simulink model "LunarMicrogrid_Full_Arch"  (R2026b)
settings: Solver=ode23t  StopTime=simulation.timeSim  MaxStep=1/(5*solarPlant.converterSwitchingFrequency)  AbsTol=1e-3
PreLoadFcn:
  | run('LunarMicrogridA_Data');
values from neighbouring files (symbols this model uses):
  Csc = Csc_cell/Ns_sc*Np_sc    (= 200)    [LunarDAB_Params.m]
  eta_sc = 0.95    [LunarDAB_Params.m]
  fsw = 100e3    (= 100000)    [LunarDAB_Params.m]
  k_restore = 1    [LunarDAB_Params.m]
  kiCurrent = 2    [LunarDAB_Params.m]
  kiVoltage = 8    [LunarDAB_Params.m]
  kpCurrent = 0.005    [LunarDAB_Params.m]
  kpVoltage = 0.4    [LunarDAB_Params.m]
  lTotal = lSeries + Llk    [LunarDAB_Params.m]
  P170_dt = 1e-4    (= 0.0001)    [P170_PV_Initialize.m]
  P170_Imp = im(ix)    [P170_PV_Initialize.m]
  P170_Vmp = vm(ix)    [P170_PV_Initialize.m]
  Rd_bat = dV_droop/Ibat_max    (= 0.232258064516)    [LunarDAB_Params.m]
  SC_enable = 1    [LunarDAB_Params.m]
  thetaIC = 0    [LunarDAB_Params.m]
  thetaMaxDab = pi/4    (= 0.785398163397)    [LunarDAB_Params.m]
  Tsw = 1/fsw    (= 1e-05)    [LunarDAB_Params.m]
  Vsc0 = sqrt((Vsc_max^2 + Vsc_min^2)/2)    [LunarDAB_Params.m]
  Vsc_max = 119    [LunarDAB_Params.m]
  Vsc_min = 66    [LunarDAB_Params.m]
undefined symbols (not defined in the file or in its folder): a_lpf_sys, battery, bms, connectedLoad, dcVoltage, DiscIntNeverNeededParam, eta_dab, Ibat_sign, mmc, Ndab, P170_T, pvDroop, sc, sensor, socLimit, solarPlant
libraries: sl_discontinuities x13, fl_lib x13, nesl_utility x13, simulink x7, batteryecm_lib x1, simulink_extras x1, ee_lib x1
(part 6 of 8)

== system LunarMicrogrid_Full_Arch/Battery + DAB + Supercap/BESS Controller/DABCtrl2/Ideal P Gain Fdbk/Internal Parameters ==
  In1 : Inport  SampleTime=SampleTime
  P Gain : Inport  Port=2  SampleTime=SampleTime
  Proportional Gain : Gain  Gain=P  ParamMin=PParamMin  ParamMax=PParamMax  OutMin=POutMin  OutMax=POutMax  RndMeth=Simplest  OutDataTypeStr=Inherit: Same as input
  Signal Specification1 : SignalSpecification  DisableCoverage=on  OutDataTypeStr=boolean  SampleTime=SampleTime
  Terminator1 : Terminator
  Out1 : Outport  SampleTime=SampleTime
  wires:
  Proportional Gain/1 -> Out1/1
  In1/1 -> Proportional Gain/1
  Signal Specification1/1 -> Terminator1/1
  P Gain/1 -> Signal Specification1/1

== system LunarMicrogrid_Full_Arch/Battery + DAB + Supercap/BESS Controller/DABCtrl2/Ideal P Gain Fdbk/Passthrough ==
  In1 : Inport  SampleTime=SampleTime
  P Gain : Inport  Port=2  SampleTime=SampleTime
  Terminator1 : Terminator
  Out1 : Outport  SampleTime=SampleTime
  wires:
  In1/1 -> Out1/1
  P Gain/1 -> Terminator1/1

== system LunarMicrogrid_Full_Arch/Battery + DAB + Supercap/BESS Controller/DABCtrl2/Integrator/Continuous ==
  U : Inport  SampleTime=SampleTime
  Reset : Inport  Port=2  SampleTime=SampleTime
  I0in : Inport  Port=3  SampleTime=SampleTime
  Ground : Ground  DisableCoverage=on
  Integrator : Integrator
  Signal Specification1 : SignalSpecification  DisableCoverage=on  OutDataTypeStr=boolean  SampleTime=SampleTime
  Terminator : Terminator
  Terminator1 : Terminator
  state : Outport  SampleTime=SampleTime
  out : Outport  Port=2  SampleTime=SampleTime
  wires:
  U/1 -> Integrator/1
  I0in/1 -> Terminator/1
  Integrator/1 -> out/1
  Ground/1 -> Signal Specification1/1
  Signal Specification1/1 -> state/1
  Reset/1 -> Terminator1/1

== system LunarMicrogrid_Full_Arch/Battery + DAB + Supercap/BESS Controller/DABCtrl2/Integrator/Disabled ==
  U : Inport  SampleTime=SampleTime
  Reset : Inport  Port=2  SampleTime=SampleTime
  I0in : Inport  Port=3  SampleTime=SampleTime
  Ground : Ground  DisableCoverage=on
  Signal Specification1 : SignalSpecification  DisableCoverage=on  OutDataTypeStr=boolean  SampleTime=SampleTime
  Signal Specification2 : SignalSpecification  DisableCoverage=on  OutDataTypeStr=boolean  SampleTime=SampleTime
  Signal Specification4 : SignalSpecification  DisableCoverage=on  OutDataTypeStr=boolean  SampleTime=SampleTime
  Terminator1 : Terminator
  Terminator2 : Terminator
  Terminator3 : Terminator
  out : Outport  SampleTime=SampleTime
  wires:
  Reset/1 -> Terminator2/1
  Signal Specification4/1 -> Terminator1/1
  I0in/1 -> Signal Specification4/1
  U/1 -> Signal Specification1/1
  Signal Specification1/1 -> Terminator3/1
  Ground/1 -> Signal Specification2/1
  Signal Specification2/1 -> out/1

== system LunarMicrogrid_Full_Arch/Battery + DAB + Supercap/BESS Controller/DABCtrl2/Integrator/Discrete ==
  U : Inport  SampleTime=SampleTime
  Reset : Inport  Port=2  SampleTime=SampleTime
  I0in : Inport  Port=3  SampleTime=SampleTime
  Ground_Integrator : Ground  DisableCoverage=on
  Integrator : DiscreteIntegrator  InitialCondition=thetaIC  SampleTime=SampleTime  OutMin=IntegratorOutMin  OutMax=IntegratorOutMax  RndMeth=Simplest  ICPrevOutput=DiscIntNeverNeededParam  ICPrevScaledInput=DiscIntNeverNeededParam
  Signal Specification1 : SignalSpecification  DisableCoverage=on  OutDataTypeStr=boolean  SampleTime=SampleTime
  Terminator : Terminator
  Terminator1 : Terminator
  Terminator2 : Terminator
  out : Outport  SampleTime=SampleTime
  state : Outport  Port=2  SampleTime=SampleTime
  wires:
  I0in/1 -> Terminator1/1
  Integrator/1 -> out/1
  U/1 -> Integrator/1
  Ground_Integrator/1 -> state/1, Signal Specification1/1
  Signal Specification1/1 -> Terminator/1
  Reset/1 -> Terminator2/1

== system LunarMicrogrid_Full_Arch/Battery + DAB + Supercap/BESS Controller/DABCtrl2/Integrator ICs/Disabled ==
  I0 : Inport  SampleTime=SampleTime
  Ground : Ground  DisableCoverage=on
  Signal Specification : SignalSpecification  DisableCoverage=on  OutDataTypeStr=boolean  SampleTime=SampleTime
  Signal Specification1 : SignalSpecification  DisableCoverage=on  OutDataTypeStr=boolean  SampleTime=SampleTime
  Terminator : Terminator
  Out1 : Outport  SampleTime=SampleTime
  wires:
  Signal Specification/1 -> Terminator/1
  I0/1 -> Signal Specification/1
  Signal Specification1/1 -> Out1/1
  Ground/1 -> Signal Specification1/1

== system LunarMicrogrid_Full_Arch/Battery + DAB + Supercap/BESS Controller/DABCtrl2/Integrator ICs/External IC ==
  I0 : Inport  SampleTime=SampleTime
  Out1 : Outport  SampleTime=SampleTime
  wires:
  I0/1 -> Out1/1

== system LunarMicrogrid_Full_Arch/Battery + DAB + Supercap/BESS Controller/DABCtrl2/Integrator ICs/Internal IC ==
  I0 : Inport  SampleTime=SampleTime
  Ground : Ground  DisableCoverage=on
  Signal Specification : SignalSpecification  DisableCoverage=on  OutDataTypeStr=boolean  SampleTime=SampleTime
  Signal Specification1 : SignalSpecification  DisableCoverage=on  OutDataTypeStr=boolean  SampleTime=SampleTime
  Terminator : Terminator
  Out1 : Outport  SampleTime=SampleTime
  wires:
  I0/1 -> Signal Specification/1
  Signal Specification/1 -> Terminator/1
  Ground/1 -> Signal Specification1/1
  Signal Specification1/1 -> Out1/1

== system LunarMicrogrid_Full_Arch/Battery + DAB + Supercap/BESS Controller/DABCtrl2/N Copy/Disabled ==
  N Gain : Inport  SampleTime=SampleTime
  Terminator : Terminator
  wires:
  N Gain/1 -> Terminator/1

== system LunarMicrogrid_Full_Arch/Battery + DAB + Supercap/BESS Controller/DABCtrl2/N Copy/Disabled wSignal Specification ==
  N Gain : Inport  SampleTime=SampleTime
  Signal Specification1 : SignalSpecification  DisableCoverage=on  OutDataTypeStr=boolean  SampleTime=SampleTime
  Terminator : Terminator
  wires:
  N Gain/1 -> Signal Specification1/1
  Signal Specification1/1 -> Terminator/1

== system LunarMicrogrid_Full_Arch/Battery + DAB + Supercap/BESS Controller/DABCtrl2/N Copy/External Parameters ==
  N Gain : Inport  SampleTime=SampleTime
  Out1 : Outport  SampleTime=SampleTime
  wires:
  N Gain/1 -> Out1/1

== system LunarMicrogrid_Full_Arch/Battery + DAB + Supercap/BESS Controller/DABCtrl2/N Copy/Internal Parameters ==
  N Gain : Inport  SampleTime=SampleTime
  N Copy : Constant  DisableCoverage=on  Value=N  OutMin=NCopyOutMin  OutMax=NCopyOutMax  OutDataTypeStr=Inherit: Inherit via back propagation  PreserveConstantTs=on
  Signal Specification : SignalSpecification  DisableCoverage=on  OutDataTypeStr=boolean  SampleTime=SampleTime
  Terminator : Terminator
  Out1 : Outport  SampleTime=SampleTime
  wires:
  N Copy/1 -> Out1/1
  N Gain/1 -> Signal Specification/1
  Signal Specification/1 -> Terminator/1

== system LunarMicrogrid_Full_Arch/Battery + DAB + Supercap/BESS Controller/DABCtrl2/N Gain/Disabled ==
  U : Inport  SampleTime=SampleTime
  N Gain : Inport  Port=2  SampleTime=SampleTime
  Signal Specification1 : SignalSpecification  DisableCoverage=on  OutDataTypeStr=boolean  SampleTime=SampleTime
  Signal Specification2 : SignalSpecification  DisableCoverage=on  OutDataTypeStr=boolean  SampleTime=SampleTime
  Terminator1 : Terminator
  Terminator2 : Terminator
  wires:
  Signal Specification2/1 -> Terminator2/1
  U/1 -> Signal Specification2/1
  N Gain/1 -> Signal Specification1/1
  Signal Specification1/1 -> Terminator1/1

== system LunarMicrogrid_Full_Arch/Battery + DAB + Supercap/BESS Controller/DABCtrl2/N Gain/External Parameters ==
  U : Inport  SampleTime=SampleTime
  N Gain : Inport  Port=2  SampleTime=SampleTime
  NProd Out : Product  OutMin=NOutMin  OutMax=NOutMax  RndMeth=Simplest  SampleTime=SampleTime
  Out1 : Outport  SampleTime=SampleTime
  wires:
  U/1 -> NProd Out/1
  N Gain/1 -> NProd Out/2
  NProd Out/1 -> Out1/1

== system LunarMicrogrid_Full_Arch/Battery + DAB + Supercap/BESS Controller/DABCtrl2/N Gain/Internal Parameters ==
  U : Inport  SampleTime=SampleTime
  N Gain : Inport  Port=2  SampleTime=SampleTime
  Filter Coefficient : Gain  Gain=N  ParamMin=NParamMin  ParamMax=NParamMax  OutMin=NOutMin  OutMax=NOutMax  RndMeth=Simplest
  Signal Specification1 : SignalSpecification  DisableCoverage=on  OutDataTypeStr=boolean  SampleTime=SampleTime
  Terminator1 : Terminator
  Out1 : Outport  SampleTime=SampleTime
  wires:
  U/1 -> Filter Coefficient/1
  Filter Coefficient/1 -> Out1/1
  N Gain/1 -> Signal Specification1/1
  Signal Specification1/1 -> Terminator1/1

== system LunarMicrogrid_Full_Arch/Battery + DAB + Supercap/BESS Controller/DABCtrl2/N Gain/Passthrough ==
  U : Inport  SampleTime=SampleTime
  N Gain : Inport  Port=2  SampleTime=SampleTime
  Terminator1 : Terminator
  Out1 : Outport  SampleTime=SampleTime
  wires:
  U/1 -> Out1/1
  N Gain/1 -> Terminator1/1

== system LunarMicrogrid_Full_Arch/Battery + DAB + Supercap/BESS Controller/DABCtrl2/P Copy/Disabled ==
  P Gain : Inport  SampleTime=SampleTime
  Terminator3 : Terminator
  wires:
  P Gain/1 -> Terminator3/1

== system LunarMicrogrid_Full_Arch/Battery + DAB + Supercap/BESS Controller/DABCtrl2/P Copy/External Parameters Ideal ==
  P Gain : Inport  SampleTime=SampleTime
  Out1 : Outport  SampleTime=SampleTime
  wires:
  P Gain/1 -> Out1/1

== system LunarMicrogrid_Full_Arch/Battery + DAB + Supercap/BESS Controller/DABCtrl2/P Copy/Internal Parameters Ideal ==
  P Gain : Inport  SampleTime=SampleTime
  P Copy : Constant  DisableCoverage=on  Value=P  OutMin=PCopyOutMin  OutMax=PCopyOutMax  OutDataTypeStr=Inherit: Inherit via back propagation  PreserveConstantTs=on
  Terminator3 : Terminator
  Out1 : Outport  SampleTime=SampleTime
  wires:
  P Copy/1 -> Out1/1
  P Gain/1 -> Terminator3/1

== system LunarMicrogrid_Full_Arch/Battery + DAB + Supercap/BESS Controller/DABCtrl2/Parallel P Gain/Disabled ==
  P Gain : Inport  SampleTime=SampleTime
  Signal Specification : SignalSpecification  DisableCoverage=on  OutDataTypeStr=boolean  SampleTime=SampleTime
  Terminator : Terminator
  wires:
  P Gain/1 -> Signal Specification/1
  Signal Specification/1 -> Terminator/1

== system LunarMicrogrid_Full_Arch/Battery + DAB + Supercap/BESS Controller/DABCtrl2/Parallel P Gain/External Parameters ==
  err : Inport  SampleTime=SampleTime
  P Gain : Inport  Port=2  SampleTime=SampleTime
  PProd Out : Product  OutMin=POutMin  OutMax=POutMax  RndMeth=Simplest  SampleTime=SampleTime  OutDataTypeStr=Inherit: Same as first input
  Out1 : Outport  SampleTime=SampleTime
  wires:
  PProd Out/1 -> Out1/1
  P Gain/1 -> PProd Out/2
  err/1 -> PProd Out/1

== system LunarMicrogrid_Full_Arch/Battery + DAB + Supercap/BESS Controller/DABCtrl2/Parallel P Gain/Internal Parameters ==
  err : Inport  SampleTime=SampleTime
  P Gain : Inport  Port=2  SampleTime=SampleTime
  Proportional Gain : Gain  Gain=P  ParamMin=PParamMin  ParamMax=PParamMax  OutMin=POutMin  OutMax=POutMax  RndMeth=Simplest  OutDataTypeStr=Inherit: Same as input
  Signal Specification : SignalSpecification  DisableCoverage=on  OutDataTypeStr=boolean  SampleTime=SampleTime
  Terminator : Terminator
  Out1 : Outport  SampleTime=SampleTime
  wires:
  Proportional Gain/1 -> Out1/1
  err/1 -> Proportional Gain/1
  Signal Specification/1 -> Terminator/1
  P Gain/1 -> Signal Specification/1

== system LunarMicrogrid_Full_Arch/Battery + DAB + Supercap/BESS Controller/DABCtrl2/Parallel P Gain/Passthrough ==
  err : Inport  SampleTime=SampleTime
  P Gain : Inport  Port=2  SampleTime=SampleTime
  Terminator : Terminator
  Out1 : Outport  SampleTime=SampleTime
  wires:
  err/1 -> Out1/1
  P Gain/1 -> Terminator/1

== system LunarMicrogrid_Full_Arch/Battery + DAB + Supercap/BESS Controller/DABCtrl2/Reset Signal/Disabled ==
  Reset : Inport  SampleTime=SampleTime
  Ground : Ground  DisableCoverage=on
  Signal Specification : SignalSpecification  DisableCoverage=on  OutDataTypeStr=boolean  SampleTime=SampleTime
  Signal Specification1 : SignalSpecification  DisableCoverage=on  OutDataTypeStr=boolean  SampleTime=SampleTime
  Terminator : Terminator
  Out1 : Outport  SampleTime=SampleTime
  wires:
  Reset/1 -> Signal Specification/1
  Signal Specification/1 -> Terminator/1
  Ground/1 -> Signal Specification1/1
  Signal Specification1/1 -> Out1/1

== system LunarMicrogrid_Full_Arch/Battery + DAB + Supercap/BESS Controller/DABCtrl2/Reset Signal/External Reset ==
  Reset : Inport  SampleTime=SampleTime
  Out1 : Outport  SampleTime=SampleTime
  wires:
  Reset/1 -> Out1/1

== system LunarMicrogrid_Full_Arch/Battery + DAB + Supercap/BESS Controller/DABCtrl2/Saturation/Enabled ==
  In1 : Inport  SampleTime=SampleTime
  Upper Limit : Inport  Port=2  SampleTime=SampleTime
  Lower Limit : Inport  Port=3  SampleTime=SampleTime
  Saturation : Saturate  UpperLimit=UpperSaturationLimit  LowerLimit=LowerSaturationLimit  LinearizeAsGain=off  SampleTime=SampleTime  OutMin=SaturationOutMin  OutMax=SaturationOutMax  OutDataTypeStr=Inherit: Inherit via back propagation  RndMeth=Simplest
  Signal Specification : SignalSpecification  DisableCoverage=on  OutDataTypeStr=boolean  SampleTime=SampleTime
  Signal Specification1 : SignalSpecification  DisableCoverage=on  OutDataTypeStr=boolean  SampleTime=SampleTime
  Terminator : Terminator
  Terminator1 : Terminator
  Out1 : Outport  SampleTime=SampleTime
  wires:
  Signal Specification1/1 -> Terminator1/1
  Upper Limit/1 -> Signal Specification/1
  Lower Limit/1 -> Signal Specification1/1
  Signal Specification/1 -> Terminator/1
  In1/1 -> Saturation/1
  Saturation/1 -> Out1/1

== system LunarMicrogrid_Full_Arch/Battery + DAB + Supercap/BESS Controller/DABCtrl2/Saturation/External ==
  In1 : Inport  SampleTime=SampleTime
  Upper Limit : Inport  Port=2  SampleTime=SampleTime
  Lower Limit : Inport  Port=3  SampleTime=SampleTime
  Saturation Dynamic : sl_discontinuities/Saturation Dynamic  OutMin=SaturationOutMin  OutMax=SaturationOutMax  OutDataTypeStr=Inherit: Same as second input  OutDataType=fixdt(1, 16)  OutScaling=2^-10  RndMeth=Simplest  DoSatur=off
  Out1 : Outport  SampleTime=SampleTime
  wires:
  Lower Limit/1 -> Saturation Dynamic/3
  Upper Limit/1 -> Saturation Dynamic/1
  Saturation Dynamic/1 -> Out1/1
  In1/1 -> Saturation Dynamic/2

== system LunarMicrogrid_Full_Arch/Battery + DAB + Supercap/BESS Controller/DABCtrl2/Saturation/Passthrough ==
  In1 : Inport  SampleTime=SampleTime
  Upper Limit : Inport  Port=2  SampleTime=SampleTime
  Lower Limit : Inport  Port=3  SampleTime=SampleTime
  Signal Specification : SignalSpecification  DisableCoverage=on  OutDataTypeStr=boolean  SampleTime=SampleTime
  Signal Specification1 : SignalSpecification  DisableCoverage=on  OutDataTypeStr=boolean  SampleTime=SampleTime
  Terminator : Terminator
  Terminator1 : Terminator
  Out1 : Outport  SampleTime=SampleTime
  wires:
  Signal Specification1/1 -> Terminator1/1
  Lower Limit/1 -> Signal Specification1/1
  Upper Limit/1 -> Signal Specification/1
  Signal Specification/1 -> Terminator/1
  In1/1 -> Out1/1

== system LunarMicrogrid_Full_Arch/Battery + DAB + Supercap/BESS Controller/DABCtrl2/Saturation Fdbk/Disabled ==
  In1 : Inport  SampleTime=SampleTime
  Signal Specification1 : SignalSpecification  DisableCoverage=on  OutDataTypeStr=boolean  SampleTime=SampleTime
  Terminator1 : Terminator
  wires:
  In1/1 -> Signal Specification1/1
  Signal Specification1/1 -> Terminator1/1

== system LunarMicrogrid_Full_Arch/Battery + DAB + Supercap/BESS Controller/DABCtrl2/Saturation Fdbk/Enabled ==
  In1 : Inport  SampleTime=SampleTime
  Saturation : Saturate  UpperLimit=UpperSaturationLimit  LowerLimit=LowerSaturationLimit  LinearizeAsGain=off  SampleTime=SampleTime  OutMin=SaturationOutMin  OutMax=SaturationOutMax  OutDataTypeStr=Inherit: Inherit via back propagation  RndMeth=Simplest
  Out1 : Outport  SampleTime=SampleTime
  wires:
  Saturation/1 -> Out1/1
  In1/1 -> Saturation/1

== system LunarMicrogrid_Full_Arch/Battery + DAB + Supercap/BESS Controller/DABCtrl2/Saturation Fdbk/External ==
  In1 : Inport  SampleTime=SampleTime
  Upper Limit : Inport  Port=2  SampleTime=SampleTime
  Lower Limit : Inport  Port=3  SampleTime=SampleTime
  Saturation Dynamic : sl_discontinuities/Saturation Dynamic  OutMin=SaturationOutMin  OutMax=SaturationOutMax  OutDataTypeStr=Inherit: Same as second input  OutDataType=fixdt(1, 16)  OutScaling=2^-10  RndMeth=Simplest  DoSatur=off
  Out1 : Outport  SampleTime=SampleTime
  wires:
  Lower Limit/1 -> Saturation Dynamic/3
  Upper Limit/1 -> Saturation Dynamic/1
  Saturation Dynamic/1 -> Out1/1
  In1/1 -> Saturation Dynamic/2

== system LunarMicrogrid_Full_Arch/Battery + DAB + Supercap/BESS Controller/DABCtrl2/Saturation Fdbk/Passthrough ==
  In1 : Inport  SampleTime=SampleTime
  Out1 : Outport  SampleTime=SampleTime
  wires:
  In1/1 -> Out1/1

== system LunarMicrogrid_Full_Arch/Battery + DAB + Supercap/BESS Controller/DABCtrl2/Sum/Passthrough_I ==
  P : Inport  SampleTime=SampleTime
  I : Inport  Port=2  SampleTime=SampleTime
  Signal Specification : SignalSpecification  OutDataTypeStr=boolean  SampleTime=SampleTime
  Terminator : Terminator
  Out1 : Outport  SampleTime=SampleTime
  wires:
  Signal Specification/1 -> Terminator/1
  P/1 -> Signal Specification/1
  I/1 -> Out1/1

== system LunarMicrogrid_Full_Arch/Battery + DAB + Supercap/BESS Controller/DABCtrl2/Sum/Passthrough_P ==
  P : Inport  SampleTime=SampleTime
  Out1 : Outport  SampleTime=SampleTime
  wires:
  P/1 -> Out1/1

== system LunarMicrogrid_Full_Arch/Battery + DAB + Supercap/BESS Controller/DABCtrl2/Sum/Sum_PD ==
  P : Inport  SampleTime=SampleTime
  D : Inport  Port=2  SampleTime=SampleTime
  Sum : Sum  Inputs=|++  OutMin=SumOutMin  OutMax=SumOutMax  RndMeth=Simplest  OutDataTypeStr=Inherit: Same as first input
  Out1 : Outport  SampleTime=SampleTime
  wires:
  P/1 -> Sum/1
  D/1 -> Sum/2
  Sum/1 -> Out1/1

== system LunarMicrogrid_Full_Arch/Battery + DAB + Supercap/BESS Controller/DABCtrl2/Sum/Sum_PI ==
  P : Inport  SampleTime=SampleTime
  I : Inport  Port=2  SampleTime=SampleTime
  Sum : Sum  Inputs=|++  OutMin=SumOutMin  OutMax=SumOutMax  RndMeth=Simplest  OutDataTypeStr=Inherit: Same as first input
  Out1 : Outport  SampleTime=SampleTime
  wires:
  I/1 -> Sum/2
  P/1 -> Sum/1
  Sum/1 -> Out1/1

== system LunarMicrogrid_Full_Arch/Battery + DAB + Supercap/BESS Controller/DABCtrl2/Sum/Sum_PID ==
  P : Inport  SampleTime=SampleTime
  I : Inport  Port=2  SampleTime=SampleTime
  D : Inport  Port=3  SampleTime=SampleTime
  Sum : Sum  Inputs=+++  OutMin=SumOutMin  OutMax=SumOutMax  RndMeth=Simplest  OutDataTypeStr=Inherit: Same as first input
  Out1 : Outport  SampleTime=SampleTime
  wires:
  I/1 -> Sum/2
  P/1 -> Sum/1
  D/1 -> Sum/3
  Sum/1 -> Out1/1

== system LunarMicrogrid_Full_Arch/Battery + DAB + Supercap/BESS Controller/DABCtrl2/Sum Fdbk/Disabled ==
  fromP : Inport  SampleTime=SampleTime
  fromState : Inport  Port=2  SampleTime=SampleTime
  fromD : Inport  Port=3  SampleTime=SampleTime
  Signal Specification1 : SignalSpecification  DisableCoverage=on  OutDataTypeStr=boolean  SampleTime=SampleTime
  Terminator1 : Terminator
  Terminator2 : Terminator
  Terminator3 : Terminator
  wires:
  fromD/1 -> Terminator3/1
  fromState/1 -> Signal Specification1/1
  fromP/1 -> Terminator1/1
  Signal Specification1/1 -> Terminator2/1

== system LunarMicrogrid_Full_Arch/Battery + DAB + Supercap/BESS Controller/DABCtrl2/Sum Fdbk/Enabled ==
  fromP : Inport  SampleTime=SampleTime
  fromState : Inport  Port=2  SampleTime=SampleTime
  fromD : Inport  Port=3  SampleTime=SampleTime
  Sum Fdbk : Sum  DisableCoverage=on  Inputs=+++  OutMin=SumOutMin  OutMax=SumOutMax  RndMeth=Simplest  OutDataTypeStr=Inherit: Same as first input
  Out1 : Outport  SampleTime=SampleTime
  wires:
  fromP/1 -> Sum Fdbk/1
  fromState/1 -> Sum Fdbk/2
  fromD/1 -> Sum Fdbk/3
  Sum Fdbk/1 -> Out1/1

== system LunarMicrogrid_Full_Arch/Battery + DAB + Supercap/BESS Controller/DABCtrl2/Sum Fdbk/Passthrough ==
  fromState : Inport  SampleTime=SampleTime
  Out1 : Outport  SampleTime=SampleTime
  wires:
  fromState/1 -> Out1/1

== system LunarMicrogrid_Full_Arch/Battery + DAB + Supercap/BESS Controller/DABCtrl2/Tracking Mode/Disabled ==
  uout : Inport  SampleTime=SampleTime
  TR : Inport  Port=2  SampleTime=SampleTime
  Signal Specification1 : SignalSpecification  DisableCoverage=on  OutDataTypeStr=boolean  SampleTime=SampleTime
  Terminator1 : Terminator
  Terminator3 : Terminator
  wires:
  uout/1 -> Terminator3/1
  TR/1 -> Signal Specification1/1
  Signal Specification1/1 -> Terminator1/1

== system LunarMicrogrid_Full_Arch/Battery + DAB + Supercap/BESS Controller/DABCtrl2/Tracking Mode/Enabled ==
  uout : Inport  SampleTime=SampleTime
  TR : Inport  Port=2  SampleTime=SampleTime
  Kt : Gain  Gain=Kt  ParamMin=KtParamMin  ParamMax=KtParamMax  OutMin=KtOutMin  OutMax=KtOutMax  RndMeth=Simplest
  SumI3 : Sum  Inputs=|-+  OutMin=SumI3OutMin  OutMax=SumI3OutMax  RndMeth=Simplest
  Out1 : Outport  SampleTime=SampleTime
  wires:
  Kt/1 -> Out1/1
  SumI3/1 -> Kt/1
  TR/1 -> SumI3/2
  uout/1 -> SumI3/1

== system LunarMicrogrid_Full_Arch/Battery + DAB + Supercap/BESS Controller/DABCtrl2/Tracking Mode Sum/Passthrough ==
  fromIgain : Inport  SampleTime=SampleTime
  fromTR : Inport  Port=2  SampleTime=SampleTime
  Signal Specification : SignalSpecification  DisableCoverage=on  OutDataTypeStr=boolean  SampleTime=SampleTime
  Terminator : Terminator
  preInt : Outport
  wires:
  fromIgain/1 -> preInt/1
  fromTR/1 -> Signal Specification/1
  Signal Specification/1 -> Terminator/1

== system LunarMicrogrid_Full_Arch/Battery + DAB + Supercap/BESS Controller/DABCtrl2/Tracking Mode Sum/Tracking Mode ==
  fromIgain : Inport  SampleTime=SampleTime
  fromTR : Inport  Port=2  SampleTime=SampleTime
  SumI1 : Sum  Inputs=|++  OutMin=SumI1OutMin  OutMax=SumI1OutMax  RndMeth=Simplest
  preInt : Outport
  wires:
  fromIgain/1 -> SumI1/1
  fromTR/1 -> SumI1/2
  SumI1/1 -> preInt/1

== system LunarMicrogrid_Full_Arch/Battery + DAB + Supercap/BESS Controller/DABCtrl2/Tsamp - Integral/Disabled ==
  U : Inport  SampleTime=SampleTime
  Ts : Inport  Port=2  SampleTime=SampleTime
  Terminator : Terminator
  Out1 : Outport  SampleTime=SampleTime
  wires:
  U/1 -> Out1/1
  Ts/1 -> Terminator/1

== system LunarMicrogrid_Full_Arch/Battery + DAB + Supercap/BESS Controller/DABCtrl2/Tsamp - Integral/External Ts ==
  U : Inport  SampleTime=SampleTime
  Ts : Inport  Port=2  SampleTime=SampleTime
  Uintegral*Ts Prod Out : Product  OutMin=UintegralTsProdOutMin  OutMax=UintegralTsProdOutMax  RndMeth=Simplest  SampleTime=SampleTime
  Out1 : Outport  SampleTime=SampleTime
  wires:
  U/1 -> Uintegral*Ts Prod Out/1
  Uintegral*Ts Prod Out/1 -> Out1/1
  Ts/1 -> Uintegral*Ts Prod Out/2

== system LunarMicrogrid_Full_Arch/Battery + DAB + Supercap/BESS Controller/DABCtrl2/Tsamp - Integral/Passthrough ==
  U : Inport  SampleTime=SampleTime
  Ts : Inport  Port=2  SampleTime=SampleTime
  Terminator : Terminator
  Out1 : Outport  SampleTime=SampleTime
  wires:
  Ts/1 -> Terminator/1
  U/1 -> Out1/1

== system LunarMicrogrid_Full_Arch/Battery + DAB + Supercap/BESS Controller/DABCtrl2/Tsamp - Integral/TsSignalSpecification ==
  U : Inport  SampleTime=SampleTime
  Ts : Inport  Port=2  SampleTime=SampleTime
  Signal Specification : SignalSpecification  DisableCoverage=on  OutDataTypeStr=boolean  SampleTime=SampleTime
  Terminator : Terminator
  Out1 : Outport  SampleTime=SampleTime
  wires:
  U/1 -> Out1/1
  Ts/1 -> Signal Specification/1
  Signal Specification/1 -> Terminator/1

== system LunarMicrogrid_Full_Arch/Battery + DAB + Supercap/BESS Controller/DABCtrl2/Tsamp - Ngain/External Ts ==
  U : Inport  SampleTime=SampleTime
  Ts : Inport  Port=2  SampleTime=SampleTime
  Ungain*Ts Prod Out : Product  OutMin=UngainTsProdOutMin  OutMax=UngainTsProdOutMax  RndMeth=Simplest  SampleTime=SampleTime
  Out1 : Outport  SampleTime=SampleTime
  wires:
  Ts/1 -> Ungain*Ts Prod Out/2
  Ungain*Ts Prod Out/1 -> Out1/1
  U/1 -> Ungain*Ts Prod Out/1

== system LunarMicrogrid_Full_Arch/Battery + DAB + Supercap/BESS Controller/DABCtrl2/Tsamp - Ngain/Passthrough ==
  U : Inport  SampleTime=SampleTime
  Ts : Inport  Port=2  SampleTime=SampleTime
  Terminator : Terminator
  Out1 : Outport  SampleTime=SampleTime
  wires:
  U/1 -> Out1/1
  Ts/1 -> Terminator/1

== system LunarMicrogrid_Full_Arch/Battery + DAB + Supercap/BESS Controller/DABCtrl2/postSat Signal/Feedback_Path ==
  feedback : Inport  SampleTime=SampleTime
  forward : Inport  Port=2  SampleTime=SampleTime
  Terminator1 : Terminator
  Out1 : Outport  SampleTime=SampleTime
  wires:
  feedback/1 -> Out1/1
  forward/1 -> Terminator1/1

== system LunarMicrogrid_Full_Arch/Battery + DAB + Supercap/BESS Controller/DABCtrl2/postSat Signal/Forward_Path ==
  feedback : Inport  SampleTime=SampleTime
  forward : Inport  Port=2  SampleTime=SampleTime
  Signal Specification1 : SignalSpecification  DisableCoverage=on  OutDataTypeStr=boolean  SampleTime=SampleTime
  Terminator1 : Terminator
  Out1 : Outport  SampleTime=SampleTime
  wires:
  forward/1 -> Out1/1
  feedback/1 -> Signal Specification1/1
  Signal Specification1/1 -> Terminator1/1

== system LunarMicrogrid_Full_Arch/Battery + DAB + Supercap/BESS Controller/DABCtrl2/preInt Signal/External PreInt ==
  preInt : Inport  SampleTime=SampleTime
  extAW : Inport  Port=2  SampleTime=SampleTime
  Terminator1 : Terminator
  Out1 : Outport  SampleTime=SampleTime
  wires:
  preInt/1 -> Terminator1/1
  extAW/1 -> Out1/1

== system LunarMicrogrid_Full_Arch/Battery + DAB + Supercap/BESS Controller/DABCtrl2/preInt Signal/Internal PreInt ==
  preInt : Inport  SampleTime=SampleTime
  extAW : Inport  Port=2  SampleTime=SampleTime
  Signal Specification1 : SignalSpecification  DisableCoverage=on  OutDataTypeStr=boolean  SampleTime=SampleTime
  Terminator1 : Terminator
  Out1 : Outport  SampleTime=SampleTime
  wires:
  Signal Specification1/1 -> Terminator1/1
  extAW/1 -> Signal Specification1/1
  preInt/1 -> Out1/1

== system LunarMicrogrid_Full_Arch/Battery + DAB + Supercap/BESS Controller/DABCtrl2/preSat Signal/Feedback_Path ==
  feedback : Inport  SampleTime=SampleTime
  forward : Inport  Port=2  SampleTime=SampleTime
  Terminator1 : Terminator
  Out1 : Outport  SampleTime=SampleTime
  wires:
  feedback/1 -> Out1/1
  forward/1 -> Terminator1/1

== system LunarMicrogrid_Full_Arch/Battery + DAB + Supercap/BESS Controller/DABCtrl2/preSat Signal/Forward_Path ==
  feedback : Inport  SampleTime=SampleTime
  forward : Inport  Port=2  SampleTime=SampleTime
  Signal Specification1 : SignalSpecification  DisableCoverage=on  OutDataTypeStr=boolean  SampleTime=SampleTime
  Terminator1 : Terminator
  Out1 : Outport  SampleTime=SampleTime
  wires:
  forward/1 -> Out1/1
  feedback/1 -> Signal Specification1/1
  Signal Specification1/1 -> Terminator1/1

== system LunarMicrogrid_Full_Arch/Battery + DAB + Supercap/BESS Controller/PIctrl/Anti-windup/Back Calculation ==
  preSat : Inport  SampleTime=SampleTime
  postSat : Inport  Port=2  SampleTime=SampleTime
  preInt : Inport  Port=3  SampleTime=SampleTime
  P : Inport  Port=4  SampleTime=SampleTime
  Kb : Gain  Gain=Kb  ParamMin=KbParamMin  ParamMax=KbParamMax  OutMin=KbOutMin  OutMax=KbOutMax  RndMeth=Simplest
  Signal Specification2 : SignalSpecification  DisableCoverage=on  OutDataTypeStr=boolean  SampleTime=SampleTime
  SumI2 : Sum  DisableCoverage=on  Inputs=|-+  OutMin=SumI2OutMin  OutMax=SumI2OutMax  RndMeth=Simplest
  SumI4 : Sum  DisableCoverage=on  Inputs=|++  OutMin=SumI4OutMin  OutMax=SumI4OutMax  RndMeth=Simplest
  Terminator2 : Terminator
  Out1 : Outport  SampleTime=SampleTime
  wires:
  preSat/1 -> SumI2/1
  postSat/1 -> SumI2/2
  SumI2/1 -> Kb/1
  Kb/1 -> SumI4/1
  SumI4/1 -> Out1/1
  preInt/1 -> SumI4/2
  Signal Specification2/1 -> Terminator2/1
  P/1 -> Signal Specification2/1

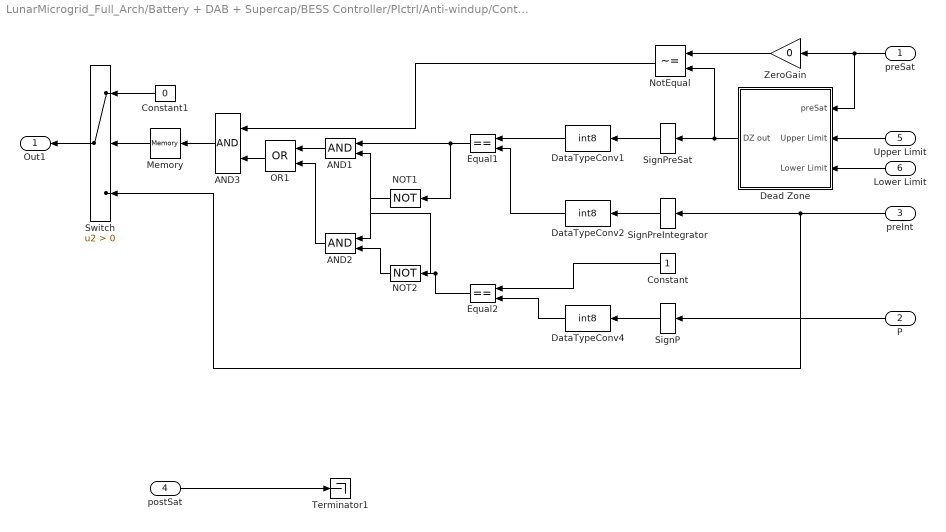
== system LunarMicrogrid_Full_Arch/Battery + DAB + Supercap/BESS Controller/PIctrl/Anti-windup/Cont. Clamping Ideal ==
  preSat : Inport  SampleTime=SampleTime
  P : Inport  Port=2  SampleTime=SampleTime
  preInt : Inport  Port=3  SampleTime=SampleTime
  postSat : Inport  Port=4  SampleTime=SampleTime
  Upper Limit : Inport  Port=5  SampleTime=SampleTime
  Lower Limit : Inport  Port=6  SampleTime=SampleTime
  AND1 : Logic  DisableCoverage=on  OutDataTypeStr=boolean
  AND2 : Logic  DisableCoverage=on  OutDataTypeStr=boolean
  AND3 : Logic  DisableCoverage=on  OutDataTypeStr=boolean
  Constant : Constant  DisableCoverage=on  OutDataTypeStr=int8  PreserveConstantTs=on
  Constant1 : Constant  DisableCoverage=on  Value=0  OutDataTypeStr=Inherit: Inherit via back propagation  PreserveConstantTs=on
  DataTypeConv1 : DataTypeConversion  DisableCoverage=on  OutDataTypeStr=int8  RndMeth=Simplest  SaturateOnIntegerOverflow=off
  DataTypeConv2 : DataTypeConversion  DisableCoverage=on  OutDataTypeStr=int8  RndMeth=Simplest  SaturateOnIntegerOverflow=off
  DataTypeConv4 : DataTypeConversion  DisableCoverage=on  OutDataTypeStr=int8  RndMeth=Simplest  SaturateOnIntegerOverflow=off
  Dead Zone : Subsystem  Variant=on  VariantControlMode=label  LabelModeActiveChoice=External  EmptyChoice=on
  Equal1 : RelationalOperator  DisableCoverage=on  Operator===  OutDataTypeStr=boolean  RndMeth=Simplest  InputSameDT=off
  Equal2 : RelationalOperator  DisableCoverage=on  Operator===  OutDataTypeStr=boolean  RndMeth=Simplest  InputSameDT=off
  Memory : Memory  DisableCoverage=on  InheritSampleTime=on
  NOT1 : Logic  DisableCoverage=on  Operator=NOT  OutDataTypeStr=boolean
  NOT2 : Logic  DisableCoverage=on  Operator=NOT  OutDataTypeStr=boolean
  NotEqual : RelationalOperator  DisableCoverage=on  Operator=~=  OutDataTypeStr=boolean  RndMeth=Simplest  InputSameDT=off
  OR1 : Logic  DisableCoverage=on  Operator=OR  OutDataTypeStr=boolean
  SignP : Signum  DisableCoverage=on
  SignPreIntegrator : Signum  DisableCoverage=on
  SignPreSat : Signum  DisableCoverage=on
  Switch : Switch  Criteria=u2 > Threshold  RndMeth=Simplest  SaturateOnIntegerOverflow=off
  Terminator1 : Terminator
  ZeroGain : Gain  DisableCoverage=on  Gain=0  RndMeth=Simplest  OutDataTypeStr=Inherit: Same as input  ParamDataTypeStr=Inherit: Same as input
  Out1 : Outport  SampleTime=SampleTime
  wires:
  Upper Limit/1 -> Dead Zone/2(Upper Limit)
  Lower Limit/1 -> Dead Zone/3(Lower Limit)
  DataTypeConv4/1 -> Equal2/2
  Constant/1 -> Equal2/1
  DataTypeConv2/1 -> Equal1/2
  DataTypeConv1/1 -> Equal1/1
  AND3/1 -> Memory/1
  OR1/1 -> AND3/2
  AND2/1 -> OR1/2
  AND1/1 -> OR1/1
  NOT2/1 -> AND2/2
  NOT1/1 -> AND2/1
  Equal2/1 -> NOT2/1, AND1/2
  Equal1/1 -> AND1/1, NOT1/1
  NotEqual/1 -> AND3/1
  SignP/1 -> DataTypeConv4/1
  SignPreIntegrator/1 -> DataTypeConv2/1
  SignPreSat/1 -> DataTypeConv1/1
  P/1 -> SignP/1
  preInt/1 -> Switch/3, SignPreIntegrator/1
  Dead Zone/1(DZ out) -> SignPreSat/1, NotEqual/2
  ZeroGain/1 -> NotEqual/1
  preSat/1 -> ZeroGain/1, Dead Zone/1(preSat)
  Switch/1 -> Out1/1
  Constant1/1 -> Switch/1
  Memory/1 -> Switch/2
  postSat/1 -> Terminator1/1

== system LunarMicrogrid_Full_Arch/Battery + DAB + Supercap/BESS Controller/PIctrl/Anti-windup/Cont. Clamping Parallel ==
  preSat : Inport  SampleTime=SampleTime
  preInt : Inport  Port=2  SampleTime=SampleTime
  postSat : Inport  Port=3  SampleTime=SampleTime
  P : Inport  Port=4  SampleTime=SampleTime
  Upper Limit : Inport  Port=5  SampleTime=SampleTime
  Lower Limit : Inport  Port=6  SampleTime=SampleTime
  AND3 : Logic  DisableCoverage=on  OutDataTypeStr=boolean
  Constant1 : Constant  DisableCoverage=on  Value=0  OutDataTypeStr=Inherit: Inherit via back propagation  PreserveConstantTs=on
  DataTypeConv1 : DataTypeConversion  DisableCoverage=on  OutDataTypeStr=int8  RndMeth=Simplest  SaturateOnIntegerOverflow=off
  DataTypeConv2 : DataTypeConversion  DisableCoverage=on  OutDataTypeStr=int8  RndMeth=Simplest  SaturateOnIntegerOverflow=off
  Dead Zone : Subsystem  Variant=on  VariantControlMode=label  LabelModeActiveChoice=External  EmptyChoice=on
  Equal1 : RelationalOperator  DisableCoverage=on  Operator===  OutDataTypeStr=boolean  RndMeth=Simplest  InputSameDT=off
  Memory : Memory  DisableCoverage=on  InheritSampleTime=on
  NotEqual : RelationalOperator  DisableCoverage=on  Operator=~=  OutDataTypeStr=boolean  RndMeth=Simplest  InputSameDT=off
  SignPreIntegrator : Signum  DisableCoverage=on
  SignPreSat : Signum  DisableCoverage=on
  Signal Specification2 : SignalSpecification  DisableCoverage=on  OutDataTypeStr=boolean  SampleTime=SampleTime
  Switch : Switch  Criteria=u2 > Threshold  RndMeth=Simplest  SaturateOnIntegerOverflow=off
  Terminator1 : Terminator
  Terminator2 : Terminator
  ZeroGain : Gain  DisableCoverage=on  Gain=0  RndMeth=Simplest  OutDataTypeStr=Inherit: Same as input  ParamDataTypeStr=Inherit: Same as input
  Out1 : Outport  SampleTime=SampleTime
  wires:
  Upper Limit/1 -> Dead Zone/2(Upper Limit)
  Lower Limit/1 -> Dead Zone/3(Lower Limit)
  AND3/1 -> Memory/1
  Constant1/1 -> Switch/1
  DataTypeConv2/1 -> Equal1/2
  DataTypeConv1/1 -> Equal1/1
  Equal1/1 -> AND3/2
  NotEqual/1 -> AND3/1
  SignPreIntegrator/1 -> DataTypeConv2/1
  SignPreSat/1 -> DataTypeConv1/1
  preInt/1 -> SignPreIntegrator/1, Switch/3
  Dead Zone/1(DZ out) -> SignPreSat/1, NotEqual/2
  ZeroGain/1 -> NotEqual/1
  preSat/1 -> ZeroGain/1, Dead Zone/1(preSat)
  Switch/1 -> Out1/1
  Memory/1 -> Switch/2
  Signal Specification2/1 -> Terminator2/1
  postSat/1 -> Terminator1/1
  P/1 -> Signal Specification2/1

== system LunarMicrogrid_Full_Arch/Battery + DAB + Supercap/BESS Controller/PIctrl/Anti-windup/Disabled ==
  preInt : Inport  SampleTime=SampleTime
  preSat : Inport  Port=2  SampleTime=SampleTime
  postSat : Inport  Port=3  SampleTime=SampleTime
  P : Inport  Port=4  SampleTime=SampleTime
  Signal Specification1 : SignalSpecification  DisableCoverage=on  OutDataTypeStr=boolean  SampleTime=SampleTime
  Signal Specification2 : SignalSpecification  DisableCoverage=on  OutDataTypeStr=boolean  SampleTime=SampleTime
  Terminator{,1..3} (4 alike) : Terminator
  wires:
  postSat/1 -> Terminator1/1
  Signal Specification2/1 -> Terminator2/1
  P/1 -> Signal Specification2/1
  preSat/1 -> Terminator/1
  preInt/1 -> Signal Specification1/1
  Signal Specification1/1 -> Terminator3/1

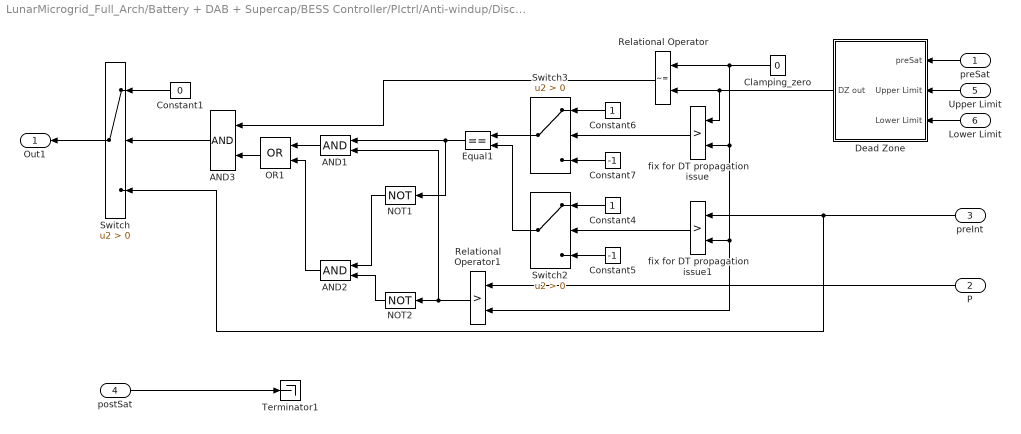
== system LunarMicrogrid_Full_Arch/Battery + DAB + Supercap/BESS Controller/PIctrl/Anti-windup/Disc. Clamping Ideal ==
  preSat : Inport  SampleTime=SampleTime
  P : Inport  Port=2  SampleTime=SampleTime
  preInt : Inport  Port=3  SampleTime=SampleTime
  postSat : Inport  Port=4  SampleTime=SampleTime
  Upper Limit : Inport  Port=5  SampleTime=SampleTime
  Lower Limit : Inport  Port=6  SampleTime=SampleTime
  AND1 : Logic  DisableCoverage=on  OutDataTypeStr=boolean
  AND2 : Logic  DisableCoverage=on  OutDataTypeStr=boolean
  AND3 : Logic  DisableCoverage=on  OutDataTypeStr=boolean
  Clamping_zero : Constant  DisableCoverage=on  Value=0  OutMin=ClampingZeroOutMin  OutMax=ClampingZeroOutMax  OutDataTypeStr=Inherit: Inherit via back propagation
  Constant1 : Constant  DisableCoverage=on  Value=0  OutDataTypeStr=Inherit: Inherit via back propagation  PreserveConstantTs=on
  Constant4 : Constant  DisableCoverage=on  OutDataTypeStr=int8
  Constant5 : Constant  DisableCoverage=on  Value=-1  OutDataTypeStr=int8
  Constant6 : Constant  DisableCoverage=on  OutDataTypeStr=int8
  Constant7 : Constant  DisableCoverage=on  Value=-1  OutDataTypeStr=int8
  Dead Zone : Subsystem  Variant=on  VariantControlMode=label  LabelModeActiveChoice=External  EmptyChoice=on
  Equal1 : RelationalOperator  DisableCoverage=on  Operator===  OutDataTypeStr=boolean  RndMeth=Simplest  InputSameDT=off
  NOT1 : Logic  DisableCoverage=on  Operator=NOT  OutDataTypeStr=boolean
  NOT2 : Logic  DisableCoverage=on  Operator=NOT  OutDataTypeStr=boolean
  OR1 : Logic  DisableCoverage=on  Operator=OR  OutDataTypeStr=boolean
  Relational Operator : RelationalOperator  DisableCoverage=on  Operator=~=  OutDataTypeStr=boolean  RndMeth=Simplest  InputSameDT=off
  Relational Operator1 : RelationalOperator  DisableCoverage=on  Operator=>  OutDataTypeStr=boolean  RndMeth=Simplest  InputSameDT=off
  Switch : Switch  Criteria=u2 > Threshold  RndMeth=Simplest  SaturateOnIntegerOverflow=off
  Switch2 : Switch  DisableCoverage=on  Criteria=u2 > Threshold  SaturateOnIntegerOverflow=off  InputSameDT=off
  Switch3 : Switch  DisableCoverage=on  Criteria=u2 > Threshold  SaturateOnIntegerOverflow=off  InputSameDT=off
  Terminator1 : Terminator
  fix for DT propagation issue : RelationalOperator  DisableCoverage=on  Operator=>  OutDataTypeStr=boolean  RndMeth=Simplest  InputSameDT=off
  fix for DT propagation issue1 : RelationalOperator  DisableCoverage=on  Operator=>  OutDataTypeStr=boolean  RndMeth=Simplest  InputSameDT=off
  Out1 : Outport  SampleTime=SampleTime
  wires:
  fix for DT propagation issue1/1 -> Switch2/2
  P/1 -> Relational Operator1/1
  Relational Operator/1 -> AND3/1
  Dead Zone/1(DZ out) -> Relational Operator/2, fix for DT propagation issue/1
  fix for DT propagation issue/1 -> Switch3/2
  Clamping_zero/1 -> fix for DT propagation issue/2, fix for DT propagation issue1/2, Relational Operator1/2, Relational Operator/1
  Switch2/1 -> Equal1/2
  Switch3/1 -> Equal1/1
  Constant7/1 -> Switch3/3
  Constant6/1 -> Switch3/1
  Constant4/1 -> Switch2/1
  Constant5/1 -> Switch2/3
  Lower Limit/1 -> Dead Zone/3(Lower Limit)
  Upper Limit/1 -> Dead Zone/2(Upper Limit)
  Switch/1 -> Out1/1
  AND3/1 -> Switch/2
  Constant1/1 -> Switch/1
  OR1/1 -> AND3/2
  AND2/1 -> OR1/2
  AND1/1 -> OR1/1
  NOT2/1 -> AND2/2
  NOT1/1 -> AND2/1
  Relational Operator1/1 -> NOT2/1, AND1/2
  Equal1/1 -> AND1/1, NOT1/1
  preInt/1 -> fix for DT propagation issue1/1, Switch/3
  preSat/1 -> Dead Zone/1(preSat)
  postSat/1 -> Terminator1/1

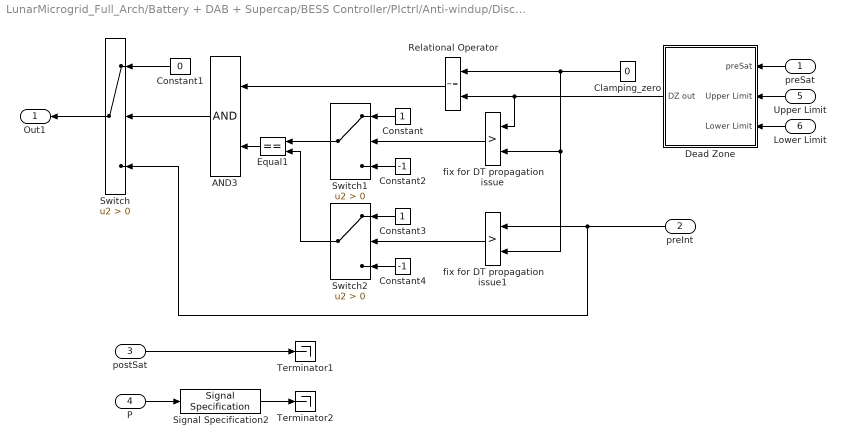
== system LunarMicrogrid_Full_Arch/Battery + DAB + Supercap/BESS Controller/PIctrl/Anti-windup/Disc. Clamping Parallel ==
  preSat : Inport  SampleTime=SampleTime
  preInt : Inport  Port=2  SampleTime=SampleTime
  postSat : Inport  Port=3  SampleTime=SampleTime
  P : Inport  Port=4  SampleTime=SampleTime
  Upper Limit : Inport  Port=5  SampleTime=SampleTime
  Lower Limit : Inport  Port=6  SampleTime=SampleTime
  AND3 : Logic  DisableCoverage=on  OutDataTypeStr=boolean
  Clamping_zero : Constant  DisableCoverage=on  Value=0  OutMin=ClampingZeroOutMin  OutMax=ClampingZeroOutMax  OutDataTypeStr=Inherit: Inherit via back propagation
  Constant : Constant  DisableCoverage=on  OutDataTypeStr=int8
  Constant1 : Constant  DisableCoverage=on  Value=0  OutDataTypeStr=Inherit: Inherit via back propagation  PreserveConstantTs=on
  Constant2 : Constant  DisableCoverage=on  Value=-1  OutDataTypeStr=int8
  Constant3 : Constant  DisableCoverage=on  OutDataTypeStr=int8
  Constant4 : Constant  DisableCoverage=on  Value=-1  OutDataTypeStr=int8
  Dead Zone : Subsystem  Variant=on  VariantControlMode=label  LabelModeActiveChoice=External  EmptyChoice=on
  Equal1 : RelationalOperator  DisableCoverage=on  Operator===  OutDataTypeStr=boolean  RndMeth=Simplest  InputSameDT=off
  Relational Operator : RelationalOperator  DisableCoverage=on  Operator=~=  OutDataTypeStr=boolean  RndMeth=Simplest  InputSameDT=off
  Signal Specification2 : SignalSpecification  DisableCoverage=on  OutDataTypeStr=boolean  SampleTime=SampleTime
  Switch : Switch  Criteria=u2 > Threshold  RndMeth=Simplest  SampleTime=SampleTime  SaturateOnIntegerOverflow=off
  Switch1 : Switch  DisableCoverage=on  Criteria=u2 > Threshold  SaturateOnIntegerOverflow=off  InputSameDT=off
  Switch2 : Switch  DisableCoverage=on  Criteria=u2 > Threshold  SaturateOnIntegerOverflow=off  InputSameDT=off
  Terminator1 : Terminator
  Terminator2 : Terminator
  fix for DT propagation issue : RelationalOperator  DisableCoverage=on  Operator=>  OutDataTypeStr=boolean  RndMeth=Simplest  InputSameDT=off
  fix for DT propagation issue1 : RelationalOperator  DisableCoverage=on  Operator=>  OutDataTypeStr=boolean  RndMeth=Simplest  InputSameDT=off
  Out1 : Outport  SampleTime=SampleTime
  wires:
  fix for DT propagation issue1/1 -> Switch2/2
  fix for DT propagation issue/1 -> Switch1/2
  Clamping_zero/1 -> fix for DT propagation issue/2, fix for DT propagation issue1/2, Relational Operator/1
  Constant1/1 -> Switch/1
  Switch2/1 -> Equal1/2
  Constant3/1 -> Switch2/1
  Constant4/1 -> Switch2/3
  Switch1/1 -> Equal1/1
  preInt/1 -> Switch/3, fix for DT propagation issue1/1
  Constant2/1 -> Switch1/3
  Constant/1 -> Switch1/1
  Relational Operator/1 -> AND3/1
  Lower Limit/1 -> Dead Zone/3(Lower Limit)
  Upper Limit/1 -> Dead Zone/2(Upper Limit)
  preSat/1 -> Dead Zone/1(preSat)
  Dead Zone/1(DZ out) -> Relational Operator/2, fix for DT propagation issue/1
  Equal1/1 -> AND3/2
  AND3/1 -> Switch/2
  Switch/1 -> Out1/1
  Signal Specification2/1 -> Terminator2/1
  postSat/1 -> Terminator1/1
  P/1 -> Signal Specification2/1

== system LunarMicrogrid_Full_Arch/Battery + DAB + Supercap/BESS Controller/PIctrl/Anti-windup/Passthrough ==
  preInt : Inport  SampleTime=SampleTime
  preSat : Inport  Port=2  SampleTime=SampleTime
  postSat : Inport  Port=3  SampleTime=SampleTime
  P : Inport  Port=4  SampleTime=SampleTime
  Signal Specification2 : SignalSpecification  DisableCoverage=on  OutDataTypeStr=boolean  SampleTime=SampleTime
  Terminator : Terminator
  Terminator1 : Terminator
  Terminator2 : Terminator
  Out1 : Outport  SampleTime=SampleTime
  wires:
  preInt/1 -> Out1/1
  preSat/1 -> Terminator/1
  postSat/1 -> Terminator1/1
  P/1 -> Signal Specification2/1
  Signal Specification2/1 -> Terminator2/1

== system LunarMicrogrid_Full_Arch/Battery + DAB + Supercap/BESS Controller/PIctrl/D Gain/Disabled ==
  D Gain : Inport  SampleTime=SampleTime
  Signal Specification : SignalSpecification  DisableCoverage=on  OutDataTypeStr=boolean  SampleTime=SampleTime
  Terminator : Terminator
  wires:
  D Gain/1 -> Signal Specification/1
  Signal Specification/1 -> Terminator/1

== system LunarMicrogrid_Full_Arch/Battery + DAB + Supercap/BESS Controller/PIctrl/D Gain/External Parameters ==
  err : Inport  SampleTime=SampleTime
  D Gain : Inport  Port=2  SampleTime=SampleTime
  DProd Out : Product  OutMin=DOutMin  OutMax=DOutMax  RndMeth=Simplest  SampleTime=SampleTime
  Out1 : Outport  SampleTime=SampleTime
  wires:
  DProd Out/1 -> Out1/1
  D Gain/1 -> DProd Out/2
  err/1 -> DProd Out/1

== system LunarMicrogrid_Full_Arch/Battery + DAB + Supercap/BESS Controller/PIctrl/D Gain/Internal Parameters ==
  err : Inport  SampleTime=SampleTime
  D Gain : Inport  Port=2  SampleTime=SampleTime
  Derivative Gain : Gain  DisableCoverage=on  Gain=D  ParamMin=DParamMin  ParamMax=DParamMax  OutMin=DOutMin  OutMax=DOutMax  RndMeth=Simplest
  Signal Specification : SignalSpecification  DisableCoverage=on  OutDataTypeStr=boolean  SampleTime=SampleTime
  Terminator : Terminator
  Out1 : Outport  SampleTime=SampleTime
  wires:
  Derivative Gain/1 -> Out1/1
  err/1 -> Derivative Gain/1
  D Gain/1 -> Signal Specification/1
  Signal Specification/1 -> Terminator/1

== system LunarMicrogrid_Full_Arch/Battery + DAB + Supercap/BESS Controller/PIctrl/External Derivative/Disabled ==
  ydot : Inport  SampleTime=SampleTime
  err : Inport  Port=2  SampleTime=SampleTime
  Signal Specification : SignalSpecification  DisableCoverage=on  OutDataTypeStr=boolean  SampleTime=SampleTime
  Terminator1 : Terminator
  Out1 : Outport  SampleTime=SampleTime
  wires:
  err/1 -> Terminator1/1
  Signal Specification/1 -> Out1/1
  ydot/1 -> Signal Specification/1

== system LunarMicrogrid_Full_Arch/Battery + DAB + Supercap/BESS Controller/PIctrl/External Derivative/Error ==
  err : Inport  SampleTime=SampleTime
  ydot : Inport  Port=2  SampleTime=SampleTime
  Signal Specification : SignalSpecification  DisableCoverage=on  OutDataTypeStr=boolean  SampleTime=SampleTime
  Terminator : Terminator
  Out1 : Outport  SampleTime=SampleTime
  wires:
  Signal Specification/1 -> Terminator/1
  ydot/1 -> Signal Specification/1
  err/1 -> Out1/1

== system LunarMicrogrid_Full_Arch/Battery + DAB + Supercap/BESS Controller/PIctrl/External Derivative/External Ydot ==
  err : Inport  SampleTime=SampleTime
  ydot : Inport  Port=2  SampleTime=SampleTime
  Terminator : Terminator
  Unary Minus : UnaryMinus
  Out1 : Outport  SampleTime=SampleTime
  wires:
  Unary Minus/1 -> Out1/1
  err/1 -> Terminator/1
  ydot/1 -> Unary Minus/1

== system LunarMicrogrid_Full_Arch/Battery + DAB + Supercap/BESS Controller/PIctrl/Filter/Cont. Filter ==
  U : Inport  SampleTime=SampleTime
  Nout : Inport  Port=2  SampleTime=SampleTime
  Reset : Inport  Port=3  SampleTime=SampleTime
  D0in : Inport  Port=4  SampleTime=SampleTime
  N : Inport  Port=5  SampleTime=SampleTime
  Ts : Inport  Port=6  SampleTime=SampleTime
  Filter : Integrator  DisableCoverage=on
  Signal Specification2 : SignalSpecification  DisableCoverage=on  OutDataTypeStr=boolean  SampleTime=SampleTime
  SumD : Sum  DisableCoverage=on  Inputs=|+-  OutMin=SumDOutMin  OutMax=SumDOutMax  RndMeth=Simplest
  Terminator{,1..3} (4 alike) : Terminator
  Y : Outport  SampleTime=SampleTime
  wires:
  Ts/1 -> Terminator3/1
  D0in/1 -> Terminator/1
  U/1 -> SumD/1
  Filter/1 -> SumD/2
  SumD/1 -> Y/1
  Nout/1 -> Filter/1
  N/1 -> Signal Specification2/1
  Signal Specification2/1 -> Terminator2/1
  Reset/1 -> Terminator1/1

== system LunarMicrogrid_Full_Arch/Battery + DAB + Supercap/BESS Controller/PIctrl/Filter/Cont. Filter Only ==
  U : Inport  SampleTime=SampleTime
  Nout : Inport  Port=2  SampleTime=SampleTime
  Reset : Inport  Port=3  SampleTime=SampleTime
  D0in : Inport  Port=4  SampleTime=SampleTime
  N : Inport  Port=5  SampleTime=SampleTime
  Ts : Inport  Port=6  SampleTime=SampleTime
  Filter : Integrator  DisableCoverage=on  InitialCondition=InitialConditionForFilter
  Signal Specification2 : SignalSpecification  DisableCoverage=on  OutDataTypeStr=boolean  SampleTime=SampleTime
  SumD : Sum  DisableCoverage=on  Inputs=|+-  OutMin=SumDOutMin  OutMax=SumDOutMax
  Terminator{,1..3} (4 alike) : Terminator
  Y : Outport  SampleTime=SampleTime
  wires:
  Nout/1 -> SumD/2
  Filter/1 -> Y/1
  SumD/1 -> Filter/1
  Ts/1 -> Terminator3/1
  D0in/1 -> Terminator/1
  U/1 -> SumD/1
  N/1 -> Signal Specification2/1
  Signal Specification2/1 -> Terminator2/1
  Reset/1 -> Terminator1/1

== system LunarMicrogrid_Full_Arch/Battery + DAB + Supercap/BESS Controller/PIctrl/Filter/Differentiator ==
  U : Inport  SampleTime=SampleTime
  Reset : Inport  Port=2  SampleTime=SampleTime
  D0in : Inport  Port=3  SampleTime=SampleTime
  Nout : Inport  Port=4  SampleTime=SampleTime
  N : Inport  Port=5  SampleTime=SampleTime
  Ts : Inport  Port=6  SampleTime=SampleTime
  DTDup : DataTypeDuplicate  NumInputPorts=3
  Diff : Sum  Inputs=+-  OutMin=DifferentiatorOutMin  OutMax=DifferentiatorOutMax  OutDataTypeStr=Inherit: Inherit via back propagation  InputSameDT=on  RndMeth=Simplest
  Signal Specification1 : SignalSpecification  DisableCoverage=on  OutDataTypeStr=boolean  SampleTime=SampleTime
  Terminator{,1..3} (4 alike) : Terminator
  Tsamp : Subsystem  Variant=on  VariantControlMode=label  LabelModeActiveChoice=InternalTs
  UD : Delay  DelayLength=1  InitialCondition=DifferentiatorICPrevScaledInput  SampleTime=SampleTime
  Y : Outport  OutMin=DifferentiatorOutMin  OutMax=DifferentiatorOutMax  SampleTime=SampleTime
  wires:
  Ts/1 -> Tsamp/2(Ts)
  D0in/1 -> Terminator/1
  U/1 -> Tsamp/1(U)
  UD/1 -> Diff/2, DTDup/3
  Tsamp/1(Out1) -> Diff/1, UD/1, DTDup/2
  Diff/1 -> Y/1, DTDup/1
  Nout/1 -> Terminator2/1
  N/1 -> Signal Specification1/1
  Signal Specification1/1 -> Terminator1/1
  Reset/1 -> Terminator3/1

== system LunarMicrogrid_Full_Arch/Battery + DAB + Supercap/BESS Controller/PIctrl/Filter/Disabled ==
  Reset : Inport  SampleTime=SampleTime
  U : Inport  Port=2  SampleTime=SampleTime
  N : Inport  Port=3  SampleTime=SampleTime
  D0in : Inport  Port=4  SampleTime=SampleTime
  Nout : Inport  Port=5  SampleTime=SampleTime
  Ts : Inport  Port=6  SampleTime=SampleTime
  Signal Specification{1..4} (4 alike) : SignalSpecification  DisableCoverage=on  OutDataTypeStr=boolean  SampleTime=SampleTime
  Terminator{1..6} (6 alike) : Terminator
  wires:
  Ts/1 -> Terminator6/1
  U/1 -> Signal Specification3/1
  Signal Specification3/1 -> Terminator3/1
  Signal Specification1/1 -> Terminator1/1
  N/1 -> Signal Specification1/1
  Nout/1 -> Signal Specification2/1
  Signal Specification4/1 -> Terminator4/1
  D0in/1 -> Signal Specification4/1
  Reset/1 -> Terminator5/1
  Signal Specification2/1 -> Terminator2/1
